simulink model "turbo_controller"  (R2025a)
settings: Solver=FixedStepAuto  StartTime=0.0  StopTime=inf  FixedStep=0.001  RelTol=1e-3
PostLoadFcn:
  | % 自动定位同目录CubeMX文件；不需要外部初始化脚本。
  | codertarget.data.setParameterValue('turbo_controller','STM32CubeMX.ProjectFile',fullfile(fileparts(get_param('turbo_controller','FileName')),'turbo_f407.ioc'));
InitFcn:
  | % 中文说明：按原控制器字段与类型创建三组接口总线；控制参数已内嵌。
  | tc_names=["EValve_Cycle" "EValve_Open" "Eblast_Cycle" "Eblast_Open" "Motor_Cycle" "Motor_Open" "EValve_Enable" "Eblast_Enable" "Motor_Enable" "SWO_Firework" "SWO_BleedAir" "EngineState" "Flag_ECUReset_Clear" "Flag_ECUReset_Save" "Flag_Reset_Enable" "Accelerator" "Nc_dem" "Nc"]; tc_types=["uint16" "uint16" "uint16" "uint16" "uint16" "uint16" "uint8" "uint8" "uint8" "uint8" "uint8" "uint8" "uint8" "uint8" "uint8" "single" "single" "single"];
  | for tc_k=1:numel(tc_names)
  |  tc_e(tc_k)=Simulink.BusElement; tc_e(tc_k).Name=char(tc_names(tc_k)); tc_e(tc_k).DataType=char(tc_types(tc_k));
  | end
  | EngineControl_Out=Simulink.Bus; EngineControl_Out.DataScope='Exported'; EngineControl_Out.Elements=tc_e;
  | clear tc_e tc_names tc_types tc_k
  | tc_names=["savedata1" "savedata2" "savedata3" "savedata4" "savedata5" "savedata6" "savedata7" "savedata8" "savedata9" "savedata10" "savedata11" "savedata12" "savedata13" "savedata14" "savedata15" "savedata16" "savedata17" "savedata18" "savedata19" "savedata20" "savedata21" "savedata22" "savedata23" "savedata24" "savedata25"]; tc_types=["single" "single" "single" "single" "single" "single" "single" "single" "single" "single" "single" "single" "single" "single" "single" "single" "single" "single" "single" "single" "single" "single" "single" "single" "single"];
  | for tc_k=1:numel(tc_names)
  |  tc_e(tc_k)=Simulink.BusElement; tc_e(tc_k).Name=char(tc_names(tc_k)); tc_e(tc_k).DataType=char(tc_types(tc_k));
  | end
  | SaveData_Out=Simulink.Bus; SaveData_Out.DataScope='Exported'; SaveData_Out.Elements=tc_e;
  | clear tc_e tc_names tc_types tc_k
  | tc_names=["senddata1" "senddata2" "senddata3" "senddata4" "senddata5" "senddata6" "senddata7" "senddata8" "senddata9" "senddata10" "senddata11" "senddata12" "senddata13" "senddata14" "senddata15" "senddata16" "senddata17" "senddata18" "senddata19" "senddata20" "senddata21" "senddata22" "senddata23" "senddata24" "senddata25" "senddata26" "senddata27" "senddata28" "senddata29"]; tc_types=["uint8" "uint8" "uint8" "uint8" "uint8" "uint8" "uint8" "uint8" "uint8" "uint8" "uint8" "uint8" "uint8" "uint8" "uint8" "uint8" "uint8" "uint8" "uint8" "uint8" "uint8" "uint8" "uint8" "uint8" "uint8" "uint8" "uint8" "uint8" "uint8"];
  | for tc_k=1:numel(tc_names)
  |  tc_e(tc_k)=Simulink.BusElement; tc_e(tc_k).Name=char(tc_names(tc_k)); tc_e(tc_k).DataType=char(tc_types(tc_k));
  | end
  | SendData_Out=Simulink.Bus; SendData_Out.DataScope='Exported'; SendData_Out.Elements=tc_e;
  | clear tc_e tc_names tc_types tc_k
  | 
  | % 以下为接口中文说明；只设置描述，不改变数值或数据类型。
  | EngineControl_Out.Description='执行控制输出（阀、电机、点火、状态及复位请求）';
  | tc_cn=["EValve_Cycle（主油阀周期计数（每计数2毫秒））" "EValve_Open（主油阀开通计数（每计数2毫秒））" "Eblast_Cycle（副油阀周期计数（每计数2毫秒））" "Eblast_Open（副油阀开通计数（每计数2毫秒））" "Motor_Cycle（起动电机周期计数）" "Motor_Open（起动电机开通计数）" "EValve_Enable（主油阀驱动使能）" "Eblast_Enable（副油阀驱动使能）" "Motor_Enable（起动电机使能）" "SWO_Firework（点火器使能（1开））" "SWO_BleedAir（引气阀使能（1开））" "EngineState（发动机状态）" "Flag_ECUReset_Clear（清除复位恢复状态请求）" "Flag_ECUReset_Save（保存复位恢复数据请求）" "Flag_Reset_Enable（处理器软件复位请求）" "Accelerator（油门／油泵给定控制量）" "Nc_dem（控制目标转速）" "Nc（发动机反馈转速（转每分））"];
  | tc_elements=EngineControl_Out.Elements;
  | for tc_k=1:numel(tc_cn)
  |  tc_elements(tc_k).Description=char(tc_cn(tc_k));
  | end
  | EngineControl_Out.Elements=tc_elements;
  | clear tc_cn tc_elements tc_k
  | SaveData_Out.Description='25项运行记录；字段含义按当前模型数据来源解释';
  | tc_cn=["savedata1（指令回显记录）" "savedata2（入口总温记录（℃））" "savedata3（电源电压记录）" "savedata4（排气温度记录（℃））" "savedata5（标定燃油压力记录）" "savedata6（副油阀占空比记录（％））" "savedata7（主油阀占空比记录（％））" "savedata8（温度修正转速记录）" "savedata9（开关输出及反馈位域）" "savedata10（物理转速记录）" "savedata11（油泵目标给定原始值）" "savedata12（起动电机占空比记录（％））" "savedata13（发动机状态码记录）" "savedata14（故障告警位域记录）" "savedata15（模型记录帧序号）" "savedata16（处理器温度记录（℃））" "savedata17（装订转速记录（沿用旧电源字段名））" "savedata18（导航高度记录）" "savedata19（飞行空速记录）" "savedata20（主阀旧记录位（恒零保留））" "savedata21（第21项保留记录（恒零））" "savedata22（保留记录项22）" "savedata23（保留记录项23）" "savedata24（保留记录项24）" "savedata25（保留记录项25）"];
  | tc_elements=SaveData_Out.Elements;
  | for tc_k=1:numel(tc_cn)
  |  tc_elements(tc_k).Description=char(tc_cn(tc_k));
  | end
  | SaveData_Out.Elements=tc_elements;
  | clear tc_cn tc_elements tc_k
  | SendData_Out.Description='29字段回传及外设命令接口；板端上位机帧只取第3至27字段';
  | tc_cn=["senddata1（回传发送允许标志（不直接上线路））" "senddata2（回传载荷长度25字节）" "senddata3（回传指令回显字节）" "senddata4（总温编码字节（℃＋80））" "senddata5（电源电压编码字节）" "senddata6（排温编码高字节）" "senddata7（排温编码低字节）" "senddata8（燃油压力编码高字节）" "senddata9（燃油压力编码低字节）" "senddata10（副油阀占空比字节（％））" "senddata11（主油阀占空比字节（％））" "senddata12（修正转速编码高字节）" "senddata13（修正转速编码低字节）" "senddata14（驱动及反馈状态位域）" "senddata15（物理转速编码高字节）" "senddata16（物理转速编码低字节）" "senddata17（油泵目标给定高字节（串口二使用））" "senddata18（油泵目标给定低字节（串口二使用））" "senddata19（起动电机占空比命令（串口一使用））" "senddata20（发动机状态码字节）" "senddata21（故障告警位域字节）" "senddata22（帧序号占位（板端另行填写））" "senddata23（处理器温度编码（℃＋50））" "senddata24（控制目标转速编码高字节）" "senddata25（控制目标转速编码低字节）" "senddata26（占位字节（板端改填实测泵速高字节））" "senddata27（占位字节（板端改填实测泵速低字节））" "senddata28（装订转速高字节（本板未发送））" "senddata29（装订转速低字节（本板未发送））"];
  | tc_elements=SendData_Out.Elements;
  | for tc_k=1:numel(tc_cn)
  |  tc_elements(tc_k).Description=char(tc_cn(tc_k));
  | end
  | SendData_Out.Elements=tc_elements;
  | clear tc_cn tc_elements tc_k
  | 
  | 
  | % FRAM模块化事务：接口类型和上电初始状态，随模型保存，无外部初始化文件。
  | clear FM_elements
  | FM_elements(1)=Simulink.BusElement;FM_elements(1).Name='phase';FM_elements(1).DataType='uint8';FM_elements(1).Dimensions=[1 1];FM_elements(1).Description='phase（当前事务阶段）';
  | FM_elements(2)=Simulink.BusElement;FM_elements(2).Name='a';FM_elements(2).DataType='uint8';FM_elements(2).Dimensions=[64 1];FM_elements(2).Description='a（启动时缓存的首区64字节）';
  | FM_elements(3)=Simulink.BusElement;FM_elements(3).Name='active';FM_elements(3).DataType='uint16';FM_elements(3).Dimensions=[1 1];FM_elements(3).Description='active（当前有效记录区地址）';
  | FM_elements(4)=Simulink.BusElement;FM_elements(4).Name='generation';FM_elements(4).DataType='uint32';FM_elements(4).Dimensions=[1 1];FM_elements(4).Description='generation（当前有效记录代号）';
  | FM_elements(5)=Simulink.BusElement;FM_elements(5).Name='record';FM_elements(5).DataType='uint8';FM_elements(5).Dimensions=[64 1];FM_elements(5).Description='record（本次冻结的待写记录）';
  | FM_elements(6)=Simulink.BusElement;FM_elements(6).Name='addr';FM_elements(6).DataType='uint16';FM_elements(6).Dimensions=[1 1];FM_elements(6).Description='addr（本次备用写入地址）';
  | FM_elements(7)=Simulink.BusElement;FM_elements(7).Name='lastSave';FM_elements(7).DataType='single';FM_elements(7).Dimensions=[1 1];FM_elements(7).Description='lastSave（上次开始保存的秒数）';
  | FM_elements(8)=Simulink.BusElement;FM_elements(8).Name='lastState';FM_elements(8).DataType='uint8';FM_elements(8).Dimensions=[1 1];FM_elements(8).Description='lastState（上次保存时的发动机状态）';
  | FM_elements(9)=Simulink.BusElement;FM_elements(9).Name='boot';FM_elements(9).DataType='boolean';FM_elements(9).Dimensions=[1 1];FM_elements(9).Description='boot（启动记录是否允许恢复）';
  | FM_elements(10)=Simulink.BusElement;FM_elements(10).Name='consumed';FM_elements(10).DataType='boolean';FM_elements(10).Dimensions=[1 1];FM_elements(10).Description='consumed（本次启动恢复通知是否已发送）';
  | FM_elements(11)=Simulink.BusElement;FM_elements(11).Name='payload';FM_elements(11).DataType='uint8';FM_elements(11).Dimensions=[20 1];FM_elements(11).Description='payload（当前20字节恢复内容）';
  | ... (+35 lines)
model workspace (MAT data in the model file):
  CRC16_Table_Reference = [0 4129 8258 12387 16516 20645 24774 28903 33032 37161 41290 45419 ... (256 elements, 256x1)]
  PE_Kaer = [0.15402 0.15402 0.12264 0.10076 0.09481 0.07601 0.07111 0.0569 0.05198 0.04926 0.05308 0.04325 ... (13 elements, 1x13)]
  PE_Nr = [21.2982 61.4260372 67.7475458 72.7394382 76.845934 80.6988798 83.8449282 86.6491912 88.9382406 89.178606 91.1938214 93.4068058 ... (13 elements, 1x13)]
  PE_Pump_Translate = 33.5999984741
  PE_RotaSpeed_Translate = 860
  PE_Taer = [0.4939154 0.4939154 0.40780982 0.34066978 0.31622756 0.30405716 0.34300244 0.26785022 0.37393554 0.23914836 0.44563948 0.31044662 ... (13 elements, 1x13)]
  PF_ACCFULLRANGE = 3360
  PF_Flag_ECUReset = 0
  PF_Flag_rx_suc = 1
  PF_Gear_Info = [40000; 45000; 50000; 55000; 57000; 59000; 60000; 61000; 61000; 61000; 61000; 61000]
  PF_K_TiaoJie = 1
  PF_Kpu = 10
  PF_MySet_Rxdata = [0 0 0 0 0 0 0 0 0 0 0 0 ... (50 elements, 50x1)]
  PF_MyUsart1_Rxdata = [0 0 0 0 0 0 0 0 0 0 0 0 ... (50 elements, 50x1)]
  PF_MyUsart2_Rxdata = [0 0 0 0 0 0 0 0 0 0 0 0 ... (50 elements, 50x1)]
  PF_Reset_Information = [0 0 0 0 0 0 0 0 0 0 0 0 ... (20 elements, 20x1)]
  PF_Sensor_X1_T4 = [0 4095]
  PF_Sensor_X2_T4 = [0 1.66666698456]
  PF_Sensor_X3_T4 = [0 504 999 1497 2010 2529 3051 3568 4076 4571 4959]
  PF_Sensor_X_P2 = [0.5 3]
  PF_Sensor_X_Poil = [0.5 3]
  PF_Sensor_X_T1t = [-50 300]
  PF_Sensor_X_Vpower = [0 3]
  PF_Sensor_X_Vpump = [0 3]
  PF_Sensor_Y1_T4 = [0 3]
  PF_Sensor_Y2_T4 = [0 5000]
  PF_Sensor_Y3_T4 = [0 100 200 300 400 500 600 700 800 900 980]
  PF_Sensor_Y_P2 = [0 1000]
  PF_Sensor_Y_Poil = [0 1000]
  PF_Sensor_Y_T1t = [-50 300]
  PF_Sensor_Y_Vpower = [0 33]
  PF_Sensor_Y_Vpump = [0 33]
  PG_CtrlMode_CloseLoop : mpt.Parameter (value not decoded)
  PG_CtrlMode_ManualAcc : mpt.Parameter (value not decoded)
  PG_CtrlMode_Origin : mpt.Parameter (value not decoded)
  PG_CtrlMode_Start : mpt.Parameter (value not decoded)
  PG_CtrlMode_Stop : mpt.Parameter (value not decoded)
  PG_ES_Clp : mpt.Parameter (value not decoded)
  PG_ES_EngStart : mpt.Parameter (value not decoded)
  PG_ES_Manual : mpt.Parameter (value not decoded)
  PG_ES_Origin : mpt.Parameter (value not decoded)
  PG_ES_Stop : mpt.Parameter (value not decoded)
  PG_Instr_BleedAirSet : mpt.Parameter (value not decoded)
  PG_Instr_CloseLoop : mpt.Parameter (value not decoded)
  PG_Instr_ECUReSet : mpt.Parameter (value not decoded)
  PG_Instr_EValveSet : mpt.Parameter (value not decoded)
  PG_Instr_EblastSet : mpt.Parameter (value not decoded)
  PG_Instr_Erase : mpt.Parameter (value not decoded)
  PG_Instr_FireWorkSet : mpt.Parameter (value not decoded)
  PG_Instr_ManualPlus : mpt.Parameter (value not decoded)
  PG_Instr_ManualrReduce : mpt.Parameter (value not decoded)
  PG_Instr_MotorSet : mpt.Parameter (value not decoded)
  PG_Instr_OilSet : mpt.Parameter (value not decoded)
  PG_Instr_SelfCheck : mpt.Parameter (value not decoded)
  PG_Instr_Start : mpt.Parameter (value not decoded)
  PG_Instr_Stop : mpt.Parameter (value not decoded)
  PG_Instr_StopZero : Simulink.Parameter (value not decoded)
  PG_Location_Air : Simulink.Parameter (value not decoded)
  PG_Location_Gnd : Simulink.Parameter (value not decoded)
  PG_ServoCtrlMode_CloseLoop : Simulink.Parameter (value not decoded)
  PG_ServoCtrlMode_CloseLoopMax : Simulink.Parameter (value not decoded)
  PG_ServoCtrlMode_CloseLoopMin : Simulink.Parameter (value not decoded)
  PG_ServoCtrlMode_ManualAcc : Simulink.Parameter (value not decoded)
  PG_ServoCtrlMode_ManualAccMax : Simulink.Parameter (value not decoded)
  PG_ServoCtrlMode_ManualAccMin : Simulink.Parameter (value not decoded)
  PG_SpeedDot_Permit : Simulink.Parameter (value not decoded)
  PL_EngineModel_Actuator = [0 10 100]
  PL_EngineModel_EngineStar_Press_P2 = [1013 1098.4 1099.144828 1099.931034 1103.613793 1162.662069 1143.793103 1131.006897 1123.186207 1117.6 1114 1111.806897 ... (127 elements, 1x127)]
  PL_EngineModel_EngineStar_RotaSpeed = [200 2000 9584 9660 10220 10240 10260 10288 10308 10368 10380 10408 ... (127 elements, 1x127)]
  PL_EngineModel_EngineStar_Temp_Exhaust = [128 129 129.1 130 131 131.1 132 133 134 134.1 135 135.1 ... (127 elements, 1x127)]
  PL_EngineModel_EngineStar_Time = [0.05 0.1 0.15 0.2 0.25 0.3 0.35 0.4 0.45 0.5 0.55 0.6 ... (127 elements, 1x127)]
  PL_EngineModel_IdleAbove_Nr = [0 21.2982 61.4260372 67.7475458 72.7394382 76.845934 80.6988798 83.8449282 86.6491912 88.9382406 89.178606 91.1938214 ... (14 elements, 1x14)]
  PL_EngineModel_IdleAbove_P2r = [0.986923266716 1.57907722675 1.81593881076 1.99358499877 2.23044658278 2.43770046879 2.65482358747 2.84233900814 3.03972366149 3.18776215149 3.25684678016 3.3950160375 ... (14 elements, 1x14)]
  PL_EngineModel_IdleAbove_Tempr = [0.0536001429337 1.07200285867 1.63301768805 1.63659103091 1.66875111667 1.72592460247 1.77595140254 1.86171163123 1.95461854565 2.03323208862 2.03323208862 2.13685903162 ... (14 elements, 1x14)]
  PL_EngineModel_IdleAbove_Ter = [0.42434128 0.42434128 0.42434128 0.30669408 0.23570008 0.22150128 0.1997974 0.23803274 0.16115638 0.24279948 0.13600422 0.31308354 ... (14 elements, 1x14)]
  PL_EngineModel_IdleAbove_Wfr = [0 10.142 23.8337 27.8905 31.9473 36.0041 40.0609 44.1177 48.1745 52.2313 52.7384 56.7952 ... (14 elements, 1x14)]
  PL_EngineModel_Press_P2 = [400 400 400 400 400 400 400 400 400 400]
  PL_EngineModel_Rotaspeed = [0 20000 96400]
  PL_EngineModel_Temp_Exhaust = [500 500 500 500 500 500 500 500 500 500]
  PL_Kaer = [0.1 0.1 0.1 0.1 0.1 0.1]
  PL_Nr = [50 60 70 80 90 100]
  PL_Taer = [0.1 0.1 0.1 0.1 0.1 0.1]
  Sig : Simulink.Signal (value not decoded)
  Ts_ms : Simulink.Parameter (value not decoded)
  false : Simulink.Parameter (value not decoded)
  true : Simulink.Parameter (value not decoded)
symbols that are objects in the model workspace (value not decoded): PG_CtrlMode_CloseLoop, PG_CtrlMode_ManualAcc, PG_CtrlMode_Origin, PG_CtrlMode_Start, PG_CtrlMode_Stop, PG_ES_Clp, PG_ES_EngStart, PG_ES_Manual, PG_ES_Origin, PG_ES_Stop, PG_Instr_BleedAirSet, PG_Instr_CloseLoop, PG_Instr_EblastSet, PG_Instr_ECUReSet, PG_Instr_Erase, PG_Instr_EValveSet, PG_Instr_FireWorkSet, PG_Instr_ManualPlus, PG_Instr_ManualrReduce, PG_Instr_MotorSet, PG_Instr_OilSet, PG_Instr_SelfCheck, PG_Instr_Start, PG_Instr_Stop, PG_Instr_StopZero, PG_ServoCtrlMode_CloseLoop, PG_ServoCtrlMode_CloseLoopMax, PG_ServoCtrlMode_CloseLoopMin, PG_ServoCtrlMode_ManualAcc, PG_ServoCtrlMode_ManualAccMax, PG_ServoCtrlMode_ManualAccMin, Ts_ms
libraries: simulink x97, stm32blockslib x10, stm32f4xxblockslib x8
(part 18 of 26)

== system turbo_controller/BoardInput_输入换算与协议解析/In03_Pump（油泵回包预留校验）/Receive（逐字节组帧与保持有效结果）_353/Step01_取字节与循环控制 ==
  note: 第一步：只处理本批收到的字节
      |
      | 接收数组最多64项，Count是这次新收到的数量，Loop给出从1开始的Index。Byte=Rx(Index)，Active=
      | (Index≤Count)。
      |
      | 处理到Index≥Count或Index=64，就把下一循环序号设65，使Loop退出；否则下一序号=Index+1。Coun
      | t=3只处理第1～3项；Count=0时仍走一次无效项保持路径，但不会把数组旧值加入帧。
      |
      | 输出Byte和Active给组帧步骤，下一序号反馈Loop。这里不识别帧头，不作CRC，不把Index当作跨批收
      | 帧位置。
  输入1_本批循环序号 : Inport
  输入2_本批有效字节数 : Inport  Port=2
  输入3_本批接收数组 : Inport  Port=3
  Active（本项在有效范围内）_242 : RelationalOperator  Operator=<=  OutDataTypeStr=boolean  RndMeth=Simplest  InputSameDT=off
  Add（加减运算）_249 : Sum  SaturateOnIntegerOverflow=on  OutDataTypeStr=Inherit: Same as first input
  AtLimit（达到处理上限）_245 : RelationalOperator  Operator===  OutDataTypeStr=boolean  RndMeth=Simplest  InputSameDT=off
  Constant（常量）_244 : Constant  Value=64  OutDataTypeStr=uint32
  Constant（常量）_247 : Constant  Value=65  OutDataTypeStr=uint32
  Constant（常量）_248 : Constant  OutDataTypeStr=uint32
  CurrentByte（按接收顺序取字节）_251 : Selector  InputPortWidth=64  IndexOptions=Index vector (port)  Indices=1  OutputSizes=1
  Last（本周期最后一项）_246 : Logic  Operator=OR  IconShape=distinctive  AllPortsSameDT=off  OutDataTypeStr=boolean
  NextIndex（处理下一项或结束）_250 : Switch  Criteria=u2 ~= 0  SaturateOnIntegerOverflow=off  InputSameDT=off
  ReceivedAll（已处理所有有效项）_243 : RelationalOperator  OutDataTypeStr=boolean  RndMeth=Simplest  InputSameDT=off
  输出1_本项字节 : Outport
  输出2_本项字节有效 : Outport  Port=2
  输出3_下一循环序号 : Outport  Port=3
  wires:
  NextIndex（处理下一项或结束）_250/1 -> 输出3_下一循环序号/1
  Active（本项在有效范围内）_242/1 -> 输出2_本项字节有效/1
  CurrentByte（按接收顺序取字节）_251/1 -> 输出1_本项字节/1
  Add（加减运算）_249/1 -> NextIndex（处理下一项或结束）_250/3
  Last（本周期最后一项）_246/1 -> NextIndex（处理下一项或结束）_250/2
  Constant（常量）_247/1 -> NextIndex（处理下一项或结束）_250/1
  AtLimit（达到处理上限）_245/1 -> Last（本周期最后一项）_246/2
  ReceivedAll（已处理所有有效项）_243/1 -> Last（本周期最后一项）_246/1
  输入3_本批接收数组/1 -> CurrentByte（按接收顺序取字节）_251/1
  Constant（常量）_244/1 -> AtLimit（达到处理上限）_245/2
  Constant（常量）_248/1 -> Add（加减运算）_249/2
  输入2_本批有效字节数/1 -> Active（本项在有效范围内）_242/2, ReceivedAll（已处理所有有效项）_243/2
  输入1_本批循环序号/1 -> Add（加减运算）_249/1, Active（本项在有效范围内）_242/1, AtLimit（达到处理上限）_245/1, ReceivedAll（已处理所有有效项）_243/1, CurrentByte（按接收顺序取字节）_251/2

== system turbo_controller/BoardInput_输入换算与协议解析/In03_Pump（油泵回包预留校验）/Receive（逐字节组帧与保持有效结果）_353/Step02_拼帧并保存半帧 ==
  note: 第二步：跨多次接收保存半帧
      |
      | 将本项字节、有效标志、上次候选缓存和上次收帧Position交给Collect。Collect识别AA55并逐项填满
      | 22字节，具体规则已在其内部再拆成五步。
      |
      | 更新后的缓存和Position经原数据类型转换，送回两条记忆块；所以第一次只收到一半，下一批还能接
      | 着填，不必从头找AA。输出候选帧与“本字节刚收齐”，交第三步校验。
      |
      | 候选缓存不等于已接受结果。即使旧缓存里已经有完整内容，没有本次收齐事件也不能再次接受它。这
      | 里的记忆按原循环节奏推进，没有增加一个额外的采样周期等待。
  输入1_本项字节 : Inport
  输入2_本项字节有效 : Inport  Port=2
  Buffer（跨周期收帧缓存）_252 : UnitDelay  InitialCondition=uint8(zeros(22,1))  SampleTime=-1  HasFrameUpgradeWarning=on
  Collect（帧头识别与缓存推进）_293 : Subsystem  Description=|
      | 逐字节组帧：本页只做“找帧头、存字节、推进位置”
      | 
      | 固定帧长为22字节，帧头是十六进制AA、55。输入为上一份候选缓存、已收字节数Position、本次Byte和本字节有效Active。输出为更新缓存、下一次使用的Position和本次收齐事件Complete。
      | 
      | Position不是本批接收数组的序号：0表示还在找AA，1表示已见AA、正在等55，2～21表示头部已确认、继续收后面的内容。跨调用的记忆由外层Step02保存，本页根据输入计算一次更新。
      | 
      | 按五步看：
      | 1 判断当前是否在等AA或55，以及字节是否匹配。
      | 2 决定这个字节应不应该进入候选缓存。
      | 3 算出本次写入位置Position+1，判断是否达到22。
      | 4 允许写入才更新对应一项，否则保留原缓存。
      | 5 按找头、重同步、收齐和无效字节规则，决定下一位置及Complete。
      | 
      | 例：AA→AA→55时，第二个AA保留继续等55的机会，不当作第二帧头写入；头确认后，后续数据即使也是AA或55，仍按普通数据收下。无效字节不推进位置，也不发收齐事件。
      | 
      | Complete仅表示候选帧刚拼满，不表示校验通过；外面的校验步骤还会检查内容。这里没有重写协议或增加等待时间，五步在同一次字节处理内完成。
  Position（已收到的字节数）_253 : UnitDelay  InitialCondition=uint16(0)  SampleTime=-1  HasFrameUpgradeWarning=on
  Store_uint16（按十六位无符号数保存状态）_536715 : DataTypeConversion  Description=为反馈回路显式指定原程序的状态类型，保持原状态更新节拍。  OutDataTypeStr=uint16  RndMeth=Round
  Store_uint8（按八位无符号数保存状态）_536714 : DataTypeConversion  Description=为反馈回路显式指定原程序的状态类型，保持原状态更新节拍。  OutDataTypeStr=uint8  RndMeth=Round
  输出1_本字节刚收齐 : Outport
  输出2_候选帧缓存 : Outport  Port=2
  wires:
  Collect（帧头识别与缓存推进）_293/3(Complete（本字节组成完整帧）_292) -> 输出1_本字节刚收齐/1  "Collect（帧头识别与缓存推进）"
  Collect（帧头识别与缓存推进）_293/1(Buffer（更新后的帧缓存）_290) -> 输出2_候选帧缓存/1, Store_uint8（按八位无符号数保存状态）_536714/1  "Collect（帧头识别与缓存推进）"
  Collect（帧头识别与缓存推进）_293/2(Position（下次接收位置）_291) -> Store_uint16（按十六位无符号数保存状态）_536715/1  "Collect（帧头识别与缓存推进）"
  Store_uint16（按十六位无符号数保存状态）_536715/1 -> Position（已收到的字节数）_253/1
  输入2_本项字节有效/1 -> Collect（帧头识别与缓存推进）_293/4(Active（当前字节有效）_257)
  输入1_本项字节/1 -> Collect（帧头识别与缓存推进）_293/3(Byte（当前字节）_256)
  Position（已收到的字节数）_253/1 -> Collect（帧头识别与缓存推进）_293/2(Position（已收字节数）_255)
  Buffer（跨周期收帧缓存）_252/1 -> Collect（帧头识别与缓存推进）_293/1(Buffer（上次收帧缓存）_254)
  Store_uint8（按八位无符号数保存状态）_536714/1 -> Buffer（跨周期收帧缓存）_252/1

== system turbo_controller/BoardInput_输入换算与协议解析/In03_Pump（油泵回包预留校验）/Receive（逐字节组帧与保持有效结果）_353/Step03_收齐且校验通过才接受 ==
  note: 第三步：刚收齐且CRC通过，才接受新帧
      |
      | Complete表示这一项字节刚把22字节补齐，先按原类型传给Verify触发校验。Verify对第6～20字节计
      | 算CRC16，分别与第21、22字节的高、低校验字节比较。
      |
      | 最后Accepted=Complete AND Verify通过。这样未收齐的数据不会被采用，Verify上一帧保留的通过状
      | 态也不会在没有新Complete时重新接收旧帧。
      |
      | CRC初值、表和覆盖范围保留原设置。校验失败只让本次Accepted为假；后面的批次统计继续看这一批
      | 有没有其他有效帧。本处不作反馈比例换算，不直接生成驱动命令。
  输入1_本字节刚收齐 : Inport
  输入2_候选帧缓存 : Inport  Port=2
  Accepted（本字节完成一帧有效数据）_345 : Logic  IconShape=distinctive  AllPortsSameDT=off  OutDataTypeStr=boolean
  Cast（数据类型转换）_343 : DataTypeConversion  OutDataTypeStr=uint32  RndMeth=Round
  Verify（完整帧校验）_344 : Subsystem  Description=|
      | 输入侧预留22字节油泵帧怎样核对CRC
      | 
      | Collect送来的是候选完整帧，本模块只在Complete有效时执行校验。内部取协议指定的待校验字节段，送CRC16逐字节计算，并取出帧尾携带的两个CRC字节。
      | 
      | 16位计算结果分为高低两部分：高字节=floor(CRC/256)，低字节=bitand(CRC,255)。分别与帧中对应位置比较，两项都一致才给出有效结果。
      | 
      | 比如计算CRC为十六进制1234，协议中的CRC高字节必须是12、低字节必须是34；顺序反过来也不能通过。CRC覆盖范围由本页Selector的固定索引决定，不应把帧头或尾部CRC自身随意加入。
      | 
      | 输出交给Receive，与“这一轮确实刚收齐一帧”共同决定是否更新反馈。不完整或校验错误时，外层保留最近有效结果。
      | 
      | 本实例CRC覆盖第6～20字节，与第21、22字节的CRC比较。
  输出1_本字节接受有效帧 : Outport
  wires:
  Accepted（本字节完成一帧有效数据）_345/1 -> 输出1_本字节接受有效帧/1
  输入2_候选帧缓存/1 -> Verify（完整帧校验）_344/2(Frame（完整候选帧）_296)
  Cast（数据类型转换）_343/1 -> Verify（完整帧校验）_344/1(Complete（完整帧执行一次）_294)
  Verify（完整帧校验）_344/1(Valid（校验是否通过）_342) -> Accepted（本字节完成一帧有效数据）_345/2  "Verify（完整帧校验）"
  输入1_本字节刚收齐/1 -> Accepted（本字节完成一帧有效数据）_345/1, Cast（数据类型转换）_343/1

== system turbo_controller/BoardInput_输入换算与协议解析/In03_Pump（油泵回包预留校验）/Receive（逐字节组帧与保持有效结果）_353/Step04_统计本批是否有有效帧 ==
  note: 第四步：统计本批有没有接受过有效帧
      |
      | 根据Loop的Index判断是不是本批第一项。第一项先把累计结果视为false，后续项继续采用Seen记忆；
      | 再把这个累计结果与本项Accepted作OR。
      |
      | 只要这一批某项收齐并校验通过，后面即使是普通字节或无效帧，批次结果仍保持true；下一批会在第
      | 一项重新统计。它不是跨所有批次永久锁存的有效标志。
      |
      | 例如本批先坏帧、后好帧，最后输出true；整批没有好帧则false。此分支只输出校验统计，不计算泵
      | 速，也没有0.875/0.125滤波，不能与BoardOutput内的实际泵反馈路径混淆。
  输入1_本字节接受有效帧 : Inport
  输入2_本批循环序号 : Inport  Port=2
  AnyValid（本次存在有效帧）_351 : Logic  Operator=OR  IconShape=distinctive  AllPortsSameDT=off  OutDataTypeStr=boolean
  BeginTick（每毫秒重新统计）_350 : Switch  Criteria=u2 ~= 0  SaturateOnIntegerOverflow=off  InputSameDT=off
  Compare（比较）_348 : RelationalOperator  Operator===  OutDataTypeStr=boolean  RndMeth=Simplest  InputSameDT=off
  Constant（常量）_347 : Constant  OutDataTypeStr=uint32
  Constant（常量）_349 : Constant  Value=false  OutDataTypeStr=boolean
  Seen（本次是否见过有效帧）_346 : UnitDelay  InitialCondition=logical(0)  SampleTime=-1  HasFrameUpgradeWarning=on
  Store_boolean（按逻辑值保存状态）_536720 : DataTypeConversion  Description=为反馈回路显式指定原程序的状态类型，保持原状态更新节拍。  OutDataTypeStr=boolean  RndMeth=Round
  输出1_本批出现过有效帧 : Outport
  wires:
  AnyValid（本次存在有效帧）_351/1 -> 输出1_本批出现过有效帧/1, Store_boolean（按逻辑值保存状态）_536720/1
  Store_boolean（按逻辑值保存状态）_536720/1 -> Seen（本次是否见过有效帧）_346/1
  Constant（常量）_347/1 -> Compare（比较）_348/2
  输入2_本批循环序号/1 -> Compare（比较）_348/1
  Seen（本次是否见过有效帧）_346/1 -> BeginTick（每毫秒重新统计）_350/3
  Compare（比较）_348/1 -> BeginTick（每毫秒重新统计）_350/2
  Constant（常量）_349/1 -> BeginTick（每毫秒重新统计）_350/1
  输入1_本字节接受有效帧/1 -> AnyValid（本次存在有效帧）_351/2
  BeginTick（每毫秒重新统计）_350/1 -> AnyValid（本次存在有效帧）_351/1

== system turbo_controller/BoardInput_输入换算与协议解析/In04_Capture（捕获间隔缓存）/Step03_计算间隔并更新环形缓存/Step01_计算回卷后的脉冲间隔 ==
  note: 第一步：把16位捕获读数换成正向间隔
      |
      | 先转换当前与上次读数的类型，避免直接用无符号数相减造成负差丢失。再计算：
      | 间隔=mod(本次Capture-上次Previous,65536)。
      |
      | 当前配置每个计数为1微秒。例：上次1000、当前2000，得到1000微秒；上次65530、当前4，得到10微
      | 秒。65536来自16位计数器的一个完整回卷周期。
      |
      | 本步骤只产生候选间隔，不检查Active，也不写缓存。回卷差分只保留模65536的结果，并没有额外累
      | 计跨越多个完整回卷的时间。
      |
      | 初始Previous沿用原模型的0，所以第一条正读数会相对0求差；本次拆分没有新增“第一脉冲只初始化
      | ”的规则。
  输入1_本项捕获读数 : Inport
  输入2_上一捕获读数 : Inport  Port=2
  Cast（数据类型转换）_382 : DataTypeConversion  OutDataTypeStr=double  RndMeth=Round
  Cast（数据类型转换）_383 : DataTypeConversion  OutDataTypeStr=double  RndMeth=Round
  Cast（数据类型转换）_387 : DataTypeConversion  OutDataTypeStr=uint32  RndMeth=Floor
  Constant（常量）_385 : Constant  Value=65536  OutDataTypeStr=double
  Difference（捕获计数差）_384 : Sum  Inputs=+-  SaturateOnIntegerOverflow=on  OutDataTypeStr=Inherit: Same as first input
  Wrap16（十六位计数回卷差分）_386 : Math  Operator=mod
  输出1_回卷后的脉冲间隔 : Outport
  wires:
  Cast（数据类型转换）_387/1 -> 输出1_回卷后的脉冲间隔/1
  Constant（常量）_385/1 -> Wrap16（十六位计数回卷差分）_386/2
  Difference（捕获计数差）_384/1 -> Wrap16（十六位计数回卷差分）_386/1
  Cast（数据类型转换）_383/1 -> Difference（捕获计数差）_384/2
  Cast（数据类型转换）_382/1 -> Difference（捕获计数差）_384/1
  Wrap16（十六位计数回卷差分）_386/1 -> Cast（数据类型转换）_387/1
  输入2_上一捕获读数/1 -> Cast（数据类型转换）_383/1
  输入1_本项捕获读数/1 -> Cast（数据类型转换）_382/1

== system turbo_controller/BoardInput_输入换算与协议解析/In04_Capture（捕获间隔缓存）/Step03_计算间隔并更新环形缓存/Step02_判断间隔是否有效 ==
  note: 第二步：决定这个间隔能否新增一条记录
      |
      | 允许保存=Active AND 间隔>0。
      |
      | Active说明本项确实属于本批新捕获，间隔>0排除重复读数。例：本次捕获和上次相同，间隔0，虽然A
      | ctive为真，也不新增间隔、不推进环形位置、不增加数量、不刷新最近有效时间。
      |
      | 没有有效新项时，即使候选差分非0，也不采用。这个许可送最后的提交步骤；本步骤自身没有记忆，
      | 也不判断转速是否超限。
  输入1_回卷后的脉冲间隔 : Inport
  输入2_本项捕获有效 : Inport  Port=2
  Constant（常量）_388 : Constant  Value=0  OutDataTypeStr=uint32
  Nonzero（零间隔丢弃）_389 : RelationalOperator  Operator=>  OutDataTypeStr=boolean  RndMeth=Simplest  InputSameDT=off
  Valid（可保存的有效间隔）_390 : Logic  IconShape=distinctive  AllPortsSameDT=off  OutDataTypeStr=boolean
  输出1_允许保存正间隔 : Outport
  wires:
  Valid（可保存的有效间隔）_390/1 -> 输出1_允许保存正间隔/1
  Nonzero（零间隔丢弃）_389/1 -> Valid（可保存的有效间隔）_390/2
  输入2_本项捕获有效/1 -> Valid（可保存的有效间隔）_390/1
  Constant（常量）_388/1 -> Nonzero（零间隔丢弃）_389/2
  输入1_回卷后的脉冲间隔/1 -> Nonzero（零间隔丢弃）_389/1

== system turbo_controller/BoardInput_输入换算与协议解析/In04_Capture（捕获间隔缓存）/Step03_计算间隔并更新环形缓存/Step03_生成缓存写入候选值 ==
  note: 第三步：准备一份只改一项的缓存候选值
      |
      | 按当前Index，把本次间隔写进旧Ring对应的位置，其余九项保留。Index是1～10的环形写入位置，不
      | 是本批捕获数组的序号。
      |
      | 例：Index=4、间隔1000，则候选数组只把第4项换成1000。即使第二步不允许保存，这里也可算出候选
      | 数组；最终会由第六步选择旧缓存，候选值不会生效。
      |
      | 这里的Assignment不增加数组长度，不求平均，也不清空其他项。
  输入1_回卷后的脉冲间隔 : Inport
  输入2_旧十项间隔缓存 : Inport  Port=2
  输入3_当前环形写入位置 : Inport  Port=3
  Cast（数据类型转换）_391 : DataTypeConversion  OutDataTypeStr=single  RndMeth=Round
  WriteRing（写入最近十个间隔）_392 : Assignment  DiagnosticForDimensions=Warning  IndexOptions=Index vector (port)  Indices=1  OutputSizes=1
  输出1_候选十项间隔缓存 : Outport
  wires:
  WriteRing（写入最近十个间隔）_392/1 -> 输出1_候选十项间隔缓存/1
  输入3_当前环形写入位置/1 -> WriteRing（写入最近十个间隔）_392/3
  Cast（数据类型转换）_391/1 -> WriteRing（写入最近十个间隔）_392/2
  输入2_旧十项间隔缓存/1 -> WriteRing（写入最近十个间隔）_392/1
  输入1_回卷后的脉冲间隔/1 -> Cast（数据类型转换）_391/1

== system turbo_controller/BoardInput_输入换算与协议解析/In04_Capture（捕获间隔缓存）/Step03_计算间隔并更新环形缓存/Step04_计算下次环形写入位置 ==
  note: 第四步：准备下一次应覆盖的环形位置
      |
      | 候选下一位置=mod(本次Index,10)+1。
      |
      | Index=1得到2，Index=9得到10，Index=10得到1。这样十项写满后继续从第1项覆盖最旧记录。
      |
      | 本步骤只算候选位置；只有第六步收到保存许可才采用它。零间隔或无效捕获不会因为这里已经算出下
      | 一位置就推进缓存。
  输入1_当前环形写入位置 : Inport
  Add（加减运算）_397 : Sum  SaturateOnIntegerOverflow=on  OutDataTypeStr=Inherit: Same as first input
  Cast（数据类型转换）_393 : DataTypeConversion  OutDataTypeStr=double  RndMeth=Round
  Constant（常量）_394 : Constant  Value=10  OutDataTypeStr=double
  Constant（常量）_396 : Constant  OutDataTypeStr=double
  Modulo（取余）_395 : Math  Operator=mod
  NextSlot（写满十项后回到第一项）_398 : DataTypeConversion  OutDataTypeStr=uint8  RndMeth=Floor
  输出1_候选下次写入位置 : Outport
  wires:
  NextSlot（写满十项后回到第一项）_398/1 -> 输出1_候选下次写入位置/1
  Add（加减运算）_397/1 -> NextSlot（写满十项后回到第一项）_398/1
  Constant（常量）_394/1 -> Modulo（取余）_395/2
  Cast（数据类型转换）_393/1 -> Modulo（取余）_395/1
  输入1_当前环形写入位置/1 -> Cast（数据类型转换）_393/1
  Constant（常量）_396/1 -> Add（加减运算）_397/2
  Modulo（取余）_395/1 -> Add（加减运算）_397/1

== system turbo_controller/BoardInput_输入换算与协议解析/In04_Capture（捕获间隔缓存）/Step03_计算间隔并更新环形缓存/Step05_计算已保存间隔数量 ==
  note: 第五步：准备累计有效间隔数量
      |
      | 候选数量=min(旧Count+1,10)。
      |
      | 未填满时，每接受一个正间隔增加1；达到10后保持10。例：旧数量8得到候选9，旧数量10仍得到10。
      | 数量到10不会让后续数据停止写入，环形位置仍继续轮转覆盖。
      |
      | 本步骤不是统计本批有几个捕获。它计算缓存有效条数的候选值，只有第六步有保存许可才提交；否则
      | 继续旧Count。
  输入1_累计有效间隔数 : Inport
  Add（加减运算）_401 : Sum  SaturateOnIntegerOverflow=on  OutDataTypeStr=Inherit: Same as first input
  Constant（常量）_399 : Constant  Value=10  OutDataTypeStr=uint8
  Constant（常量）_400 : Constant  OutDataTypeStr=uint8
  Filled（有效个数最多十项）_402 : MinMax  Inputs=2
  输出1_候选有效间隔数量 : Outport
  wires:
  Filled（有效个数最多十项）_402/1 -> 输出1_候选有效间隔数量/1
  Add（加减运算）_401/1 -> Filled（有效个数最多十项）_402/2
  Constant（常量）_399/1 -> Filled（有效个数最多十项）_402/1
  Constant（常量）_400/1 -> Add（加减运算）_401/2
  输入1_累计有效间隔数/1 -> Add（加减运算）_401/1

== system turbo_controller/BoardInput_输入换算与协议解析/In04_Capture（捕获间隔缓存）/Step03_计算间隔并更新环形缓存/Step06_有效才提交并更新时间 ==
  note: 第六步：按许可提交候选状态，并记录新鲜程度
      |
      | 分别选择两类状态：
      | Previous：Active为真就采用当前Capture，否则保持旧Previous。
      | Ring、Index、Count、LastTime：只有第二步允许保存时，才采用第三～五步候选值，并把LastTime更
      | 新为当前Seconds；否则全部保持旧值。
      |
      | 例：有效捕获但与上次相同，Previous仍更新到当前读数，其他四项不变。这种情况下不会伪造一条0
      | 间隔，也不会让后面的超时判断误以为又收到了一条有效间隔。
      |
      | LastTime记录的是本批处理时刻，单位秒；同一批多个捕获共用这一时刻。它不等同于每个脉冲精确的
      | 硬件到达时刻，精确间隔来自计数差分。
      |
      | 五项输出交外层记忆。本处没有新增延迟，没有直接输出转速，也不负责选择电机反馈或捕获测速。
  输入1_本项捕获读数 : Inport
  输入2_当前处理时刻_秒 : Inport  Port=2
  输入3_本项捕获有效 : Inport  Port=3
  输入4_上一捕获读数 : Inport  Port=4
  输入5_候选十项间隔缓存 : Inport  Port=5
  输入6_允许保存正间隔 : Inport  Port=6
  输入7_旧十项间隔缓存 : Inport  Port=7
  输入8_候选下次写入位置 : Inport  Port=8
  输入9_当前环形写入位置 : Inport  Port=9
  输入10_候选有效间隔数量 : Inport  Port=10
  输入11_累计有效间隔数 : Inport  Port=11
  输入12_上次有效间隔时刻 : Inport  Port=12
  Cast（数据类型转换）_403 : DataTypeConversion  OutDataTypeStr=uint32  RndMeth=Round
  Cast（数据类型转换）_412 : DataTypeConversion  OutDataTypeStr=single  RndMeth=Round
  Select（按条件选择）_{404,406,408,410,413} (5 alike) : Switch  Criteria=u2 ~= 0  SaturateOnIntegerOverflow=off  InputSameDT=off
  输出1_下一差分基准 : Outport
  输出2_更新后的十项间隔 : Outport  Port=2
  输出3_下一环形写入位置 : Outport  Port=3
  输出4_更新后的有效间隔数 : Outport  Port=4
  输出5_最近有效间隔处理时刻 : Outport  Port=5
  wires:
  输入1_本项捕获读数/1 -> Cast（数据类型转换）_403/1
  输入2_当前处理时刻_秒/1 -> Cast（数据类型转换）_412/1
  Cast（数据类型转换）_403/1 -> Select（按条件选择）_404/1
  输入3_本项捕获有效/1 -> Select（按条件选择）_404/2
  输入4_上一捕获读数/1 -> Select（按条件选择）_404/3
  输入9_当前环形写入位置/1 -> Select（按条件选择）_408/3
  输入5_候选十项间隔缓存/1 -> Select（按条件选择）_406/1
  Select（按条件选择）_406/1 -> 输出2_更新后的十项间隔/1
  输入11_累计有效间隔数/1 -> Select（按条件选择）_410/3
  输入7_旧十项间隔缓存/1 -> Select（按条件选择）_406/3
  Cast（数据类型转换）_412/1 -> Select（按条件选择）_413/1
  Select（按条件选择）_404/1 -> 输出1_下一差分基准/1
  输入12_上次有效间隔时刻/1 -> Select（按条件选择）_413/3
  输入10_候选有效间隔数量/1 -> Select（按条件选择）_410/1
  输入6_允许保存正间隔/1 -> Select（按条件选择）_410/2, Select（按条件选择）_408/2, Select（按条件选择）_413/2, Select（按条件选择）_406/2
  输入8_候选下次写入位置/1 -> Select（按条件选择）_408/1
  Select（按条件选择）_413/1 -> 输出5_最近有效间隔处理时刻/1
  Select（按条件选择）_408/1 -> 输出3_下一环形写入位置/1
  Select（按条件选择）_410/1 -> 输出4_更新后的有效间隔数/1

== system turbo_controller/BoardInput_输入换算与协议解析/In05_Speed（转速来源选择与滤波）/CaptureSpeed（去极值估算转速）_19/Step01_选出有效间隔 ==
  note: 第一步：标出前n个有效位置，求和时把其他位置变0
      |
      | 缓存固定十项，但刚开始未必填满。将序号1～10分别与Count比较，序号≤Count才标记为有效。
      |
      | 求和用的数组：有效位置保留原间隔，无效位置填0。与此同时把有效位置掩码送下一步，用于寻找真
      | 正有效项中的最大值和最小值。
      |
      | 例：Count=3，缓存[1000,1100,900,0,…]，求和数组只采用前三项，后七项不作为测量。Count是间隔
      | 条数，不是时间，也不是每转脉冲数。
      |
      | 本步骤不改写原缓存，只生成本次计算用的数据与掩码。
  输入1_有效间隔条数 : Inport
  输入2_原十项间隔缓存 : Inport  Port=2
  Cast（数据类型转换）_447 : DataTypeConversion  OutDataTypeStr=uint32  RndMeth=Round
  Constant（常量）_449 : Constant  Value=zeros(10,1)  OutDataTypeStr=single
  Indices（十项缓存的序号）_446 : Constant  Value=(1:10)'  OutDataTypeStr=uint32
  ValidSlots（只用前面有效的项）_448 : RelationalOperator  Operator=<=  OutDataTypeStr=boolean  RndMeth=Simplest  InputSameDT=off
  ValidValues（无效项按零参加求和）_450 : Switch  Criteria=u2 ~= 0  SaturateOnIntegerOverflow=off  InputSameDT=off
  输出1_有效位置掩码 : Outport
  输出2_无效项已清零的求和数据 : Outport  Port=2
  wires:
  ValidValues（无效项按零参加求和）_450/1 -> 输出2_无效项已清零的求和数据/1
  Constant（常量）_449/1 -> ValidValues（无效项按零参加求和）_450/3
  ValidSlots（只用前面有效的项）_448/1 -> 输出1_有效位置掩码/1, ValidValues（无效项按零参加求和）_450/2
  输入2_原十项间隔缓存/1 -> ValidValues（无效项按零参加求和）_450/1
  Cast（数据类型转换）_447/1 -> ValidSlots（只用前面有效的项）_448/2
  Indices（十项缓存的序号）_446/1 -> ValidSlots（只用前面有效的项）_448/1
  输入1_有效间隔条数/1 -> Cast（数据类型转换）_447/1

== system turbo_controller/BoardInput_输入换算与协议解析/In05_Speed（转速来源选择与滤波）/CaptureSpeed（去极值估算转速）_19/Step02_去掉最大最小再求和 ==
  note: 第二步：去掉一个最大间隔和一个最小间隔
      |
      | 先对第一步的求和数组求总和。找最大值时，无效位置用0占位；找最小值时，无效位置用single最大
      | 有限值占位，避免未填满缓存的0被误当作最小有效间隔。
      |
      | S=有效间隔总和-最大有效间隔-最小有效间隔。
      | 例：[900,1000,1100]的总和3000，去掉1100和900，S=1000；剩下一项用于估速。若十项都是1000，去
      | 掉其中两项，S=8000。
      |
      | 每种极值只减一项；即使有多个相同最大值，也不是全部删除。这里求的是剩余间隔总和，还没有除以
      | n-2；第四步会把剩余项数并入转速公式。
  输入1_原十项间隔缓存 : Inport
  输入2_有效位置掩码 : Inport  Port=2
  输入3_无效项已清零的求和数据 : Inport  Port=3
  Constant（常量）_452 : Constant  Value=0  OutDataTypeStr=single
  Constant（常量）_455 : Constant  Value=realmax('single')  OutDataTypeStr=single
  Maximum（去掉一个最大间隔）_454 : MinMax  Function=max
  Minimum（去掉一个最小间隔）_457 : MinMax
  Select（按条件选择）_453 : Switch  Criteria=u2 ~= 0  SaturateOnIntegerOverflow=off  InputSameDT=off
  Select（按条件选择）_456 : Switch  Criteria=u2 ~= 0  SaturateOnIntegerOverflow=off  InputSameDT=off
  Sum（有效间隔总和）_451 : Sum  Inputs=+  OutDataTypeStr=single  AccumDataTypeStr=single
  TrimmedSum（去掉一个最大值和一个最小值）_458 : Sum  Inputs=+--  SaturateOnIntegerOverflow=on  OutDataTypeStr=Inherit: Same as first input
  输出1_去极值后间隔总和 : Outport
  wires:
  输入1_原十项间隔缓存/1 -> Select（按条件选择）_453/1, Select（按条件选择）_456/1
  输入2_有效位置掩码/1 -> Select（按条件选择）_456/2, Select（按条件选择）_453/2
  Constant（常量）_452/1 -> Select（按条件选择）_453/3
  Constant（常量）_455/1 -> Select（按条件选择）_456/3
  输入3_无效项已清零的求和数据/1 -> Sum（有效间隔总和）_451/1
  Select（按条件选择）_453/1 -> Maximum（去掉一个最大间隔）_454/1
  Select（按条件选择）_456/1 -> Minimum（去掉一个最小间隔）_457/1
  Sum（有效间隔总和）_451/1 -> TrimmedSum（去掉一个最大值和一个最小值）_458/1
  Maximum（去掉一个最大间隔）_454/1 -> TrimmedSum（去掉一个最大值和一个最小值）_458/2
  TrimmedSum（去掉一个最大值和一个最小值）_458/1 -> 输出1_去极值后间隔总和/1
  Minimum（去掉一个最小间隔）_457/1 -> TrimmedSum（去掉一个最大值和一个最小值）_458/3

== system turbo_controller/BoardInput_输入换算与协议解析/In05_Speed（转速来源选择与滤波）/CaptureSpeed（去极值估算转速）_19/Step03_检查分母并防止除零 ==
  note: 第三步：判断去极值后的总和能否作分母
      |
      | Valid=(S>0)。有效时把S交给下一步；无效时，内部改用1作为安全分母，避免除零。
      |
      | 安全分母1只是防止算术错误，不能表示测量间隔为1微秒。Valid为假时，后面的数值输出不可单独当
      | 作有效转速。
      |
      | 本步骤也不判断Count≥3。这个数量条件在外层Status；只有数量、分母和时间条件都满足，外层才会
      | 采用捕获估速。
  输入1_去极值后间隔总和 : Inport
  Constant（常量）_459 : Constant  Value=0  OutDataTypeStr=single
  Constant（常量）_461 : Constant  OutDataTypeStr=single
  Positive（分母必须大于零）_460 : RelationalOperator  Operator=>  OutDataTypeStr=boolean  RndMeth=Simplest  InputSameDT=off
  SafeDenominator（无效时避免除零）_462 : Switch  Criteria=u2 ~= 0  SaturateOnIntegerOverflow=off  InputSameDT=off
  输出1_用于计算的安全分母 : Outport
  输出2_分母为正 : Outport  Port=2
  wires:
  SafeDenominator（无效时避免除零）_462/1 -> 输出1_用于计算的安全分母/1
  Constant（常量）_461/1 -> SafeDenominator（无效时避免除零）_462/3
  Positive（分母必须大于零）_460/1 -> SafeDenominator（无效时避免除零）_462/2, 输出2_分母为正/1
  Constant（常量）_459/1 -> Positive（分母必须大于零）_460/2
  输入1_去极值后间隔总和/1 -> SafeDenominator（无效时避免除零）_462/1, Positive（分母必须大于零）_460/1

== system turbo_controller/BoardInput_输入换算与协议解析/In05_Speed（转速来源选择与滤波）/CaptureSpeed（去极值估算转速）_19/Step04_按每转三脉冲计算转速 ==
  note: 第四步：将剩余间隔总和换算成每分钟转数
      |
      | 输入有效间隔数n与前一步给出的安全分母S。先求剩余条数n-2，再计算：
      | 转速=60000000×(n-2)/(3×S)。
      |
      | 60000000是一分钟的微秒数；3表示本工程每转3个脉冲；S/(n-2)相当于去极值后的平均脉冲间隔。这
      | 里没有另外的隐含乘100或除100。
      |
      | 例：n=10、S=8000微秒，得到20000转/分。这个数是捕获候选转速，最终仍由外层的数量判断、超时判
      | 断和来源选择决定是否使用。不能因为采用了安全分母就忽略Valid。
  输入1_有效间隔条数 : Inport
  输入2_用于计算的安全分母 : Inport  Port=2
  Add（加减运算）_466 : Sum  Inputs=+-  SaturateOnIntegerOverflow=on  OutDataTypeStr=Inherit: Same as first input
  Cast（数据类型转换）_464 : DataTypeConversion  OutDataTypeStr=single  RndMeth=Round
  Constant（常量）_463 : Constant  Value=60000000  OutDataTypeStr=single
  Constant（常量）_465 : Constant  Value=2  OutDataTypeStr=single
  Constant（常量）_468 : Constant  Value=3  OutDataTypeStr=single
  Numerator（每分钟微秒数乘剩余间隔数）_467 : Product  Inputs=**  SaturateOnIntegerOverflow=on  OutDataTypeStr=Inherit: Same as first input
  Pulses（每转三个脉冲）_469 : Product  Inputs=**  SaturateOnIntegerOverflow=on  OutDataTypeStr=Inherit: Same as first input
  Speed（去极值估算的转速）_470 : Product  Inputs=*/  SaturateOnIntegerOverflow=on  OutDataTypeStr=Inherit: Same as first input
  输出1_捕获候选转速_RPM : Outport
  wires:
  Speed（去极值估算的转速）_470/1 -> 输出1_捕获候选转速_RPM/1
  Pulses（每转三个脉冲）_469/1 -> Speed（去极值估算的转速）_470/2
  Numerator（每分钟微秒数乘剩余间隔数）_467/1 -> Speed（去极值估算的转速）_470/1
  Constant（常量）_468/1 -> Pulses（每转三个脉冲）_469/2
  输入2_用于计算的安全分母/1 -> Pulses（每转三个脉冲）_469/1
  Add（加减运算）_466/1 -> Numerator（每分钟微秒数乘剩余间隔数）_467/2
  Constant（常量）_463/1 -> Numerator（每分钟微秒数乘剩余间隔数）_467/1
  输入1_有效间隔条数/1 -> Cast（数据类型转换）_464/1
  Constant（常量）_465/1 -> Add（加减运算）_466/2
  Cast（数据类型转换）_464/1 -> Add（加减运算）_466/1

== system turbo_controller/BoardOutput_串口封装与阀门时序/Out01_Pump（泵反馈解析与滤波）/Receive（逐字节组帧与保持有效结果）_680/Step01_取字节与循环控制 ==
  note: 第一步：只处理本批收到的字节
      |
      | 接收数组最多64项，Count是这次新收到的数量，Loop给出从1开始的Index。Byte=Rx(Index)，Active=
      | (Index≤Count)。
      |
      | 处理到Index≥Count或Index=64，就把下一循环序号设65，使Loop退出；否则下一序号=Index+1。Coun
      | t=3只处理第1～3项；Count=0时仍走一次无效项保持路径，但不会把数组旧值加入帧。
      |
      | 输出Byte和Active给组帧步骤，下一序号反馈Loop。这里不识别帧头，不作CRC，不把Index当作跨批收
      | 帧位置。
  输入1_本批循环序号 : Inport
  输入2_本批有效字节数 : Inport  Port=2
  输入3_本批接收数组 : Inport  Port=3
  Active（本项在有效范围内）_560 : RelationalOperator  Operator=<=  OutDataTypeStr=boolean  RndMeth=Simplest  InputSameDT=off
  Add（加减运算）_567 : Sum  SaturateOnIntegerOverflow=on  OutDataTypeStr=Inherit: Same as first input
  AtLimit（达到处理上限）_563 : RelationalOperator  Operator===  OutDataTypeStr=boolean  RndMeth=Simplest  InputSameDT=off
  Constant（常量）_562 : Constant  Value=64  OutDataTypeStr=uint32
  Constant（常量）_565 : Constant  Value=65  OutDataTypeStr=uint32
  Constant（常量）_566 : Constant  OutDataTypeStr=uint32
  CurrentByte（按接收顺序取字节）_569 : Selector  InputPortWidth=64  IndexOptions=Index vector (port)  Indices=1  OutputSizes=1
  Last（本周期最后一项）_564 : Logic  Operator=OR  IconShape=distinctive  AllPortsSameDT=off  OutDataTypeStr=boolean
  NextIndex（处理下一项或结束）_568 : Switch  Criteria=u2 ~= 0  SaturateOnIntegerOverflow=off  InputSameDT=off
  ReceivedAll（已处理所有有效项）_561 : RelationalOperator  OutDataTypeStr=boolean  RndMeth=Simplest  InputSameDT=off
  输出1_本项字节 : Outport
  输出2_本项字节有效 : Outport  Port=2
  输出3_下一循环序号 : Outport  Port=3
  wires:
  NextIndex（处理下一项或结束）_568/1 -> 输出3_下一循环序号/1
  Active（本项在有效范围内）_560/1 -> 输出2_本项字节有效/1
  CurrentByte（按接收顺序取字节）_569/1 -> 输出1_本项字节/1
  Add（加减运算）_567/1 -> NextIndex（处理下一项或结束）_568/3
  Last（本周期最后一项）_564/1 -> NextIndex（处理下一项或结束）_568/2
  Constant（常量）_565/1 -> NextIndex（处理下一项或结束）_568/1
  AtLimit（达到处理上限）_563/1 -> Last（本周期最后一项）_564/2
  ReceivedAll（已处理所有有效项）_561/1 -> Last（本周期最后一项）_564/1
  输入3_本批接收数组/1 -> CurrentByte（按接收顺序取字节）_569/1
  Constant（常量）_562/1 -> AtLimit（达到处理上限）_563/2
  Constant（常量）_566/1 -> Add（加减运算）_567/2
  输入2_本批有效字节数/1 -> ReceivedAll（已处理所有有效项）_561/2, Active（本项在有效范围内）_560/2
  输入1_本批循环序号/1 -> Active（本项在有效范围内）_560/1, Add（加减运算）_567/1, AtLimit（达到处理上限）_563/1, CurrentByte（按接收顺序取字节）_569/2, ReceivedAll（已处理所有有效项）_561/1

== system turbo_controller/BoardOutput_串口封装与阀门时序/Out01_Pump（泵反馈解析与滤波）/Receive（逐字节组帧与保持有效结果）_680/Step02_拼帧并保存半帧 ==
  note: 第二步：跨多次接收保存半帧
      |
      | 将本项字节、有效标志、上次候选缓存和上次收帧Position交给Collect。Collect识别AA55并逐项填满
      | 22字节，具体规则已在其内部再拆成五步。
      |
      | 更新后的缓存和Position经原数据类型转换，送回两条记忆块；所以第一次只收到一半，下一批还能接
      | 着填，不必从头找AA。输出候选帧与“本字节刚收齐”，交第三步校验。
      |
      | 候选缓存不等于已接受结果。即使旧缓存里已经有完整内容，没有本次收齐事件也不能再次接受它。这
      | 里的记忆按原循环节奏推进，没有增加一个额外的采样周期等待。
  输入1_本项字节 : Inport
  输入2_本项字节有效 : Inport  Port=2
  Buffer（跨周期收帧缓存）_570 : UnitDelay  InitialCondition=uint8(zeros(22,1))  SampleTime=-1  HasFrameUpgradeWarning=on
  Collect（帧头识别与缓存推进）_611 : Subsystem  Description=|
      | 逐字节组帧：本页只做“找帧头、存字节、推进位置”
      | 
      | 固定帧长为22字节，帧头是十六进制AA、55。输入为上一份候选缓存、已收字节数Position、本次Byte和本字节有效Active。输出为更新缓存、下一次使用的Position和本次收齐事件Complete。
      | 
      | Position不是本批接收数组的序号：0表示还在找AA，1表示已见AA、正在等55，2～21表示头部已确认、继续收后面的内容。跨调用的记忆由外层Step02保存，本页根据输入计算一次更新。
      | 
      | 按五步看：
      | 1 判断当前是否在等AA或55，以及字节是否匹配。
      | 2 决定这个字节应不应该进入候选缓存。
      | 3 算出本次写入位置Position+1，判断是否达到22。
      | 4 允许写入才更新对应一项，否则保留原缓存。
      | 5 按找头、重同步、收齐和无效字节规则，决定下一位置及Complete。
      | 
      | 例：AA→AA→55时，第二个AA保留继续等55的机会，不当作第二帧头写入；头确认后，后续数据即使也是AA或55，仍按普通数据收下。无效字节不推进位置，也不发收齐事件。
      | 
      | Complete仅表示候选帧刚拼满，不表示校验通过；外面的校验步骤还会检查内容。这里没有重写协议或增加等待时间，五步在同一次字节处理内完成。
  Position（已收到的字节数）_571 : UnitDelay  InitialCondition=uint16(0)  SampleTime=-1  HasFrameUpgradeWarning=on
  Store_uint16（按十六位无符号数保存状态）_537039 : DataTypeConversion  Description=为反馈回路显式指定原程序的状态类型，保持原状态更新节拍。  OutDataTypeStr=uint16  RndMeth=Round
  Store_uint8（按八位无符号数保存状态）_537038 : DataTypeConversion  Description=为反馈回路显式指定原程序的状态类型，保持原状态更新节拍。  OutDataTypeStr=uint8  RndMeth=Round
  输出1_本字节刚收齐 : Outport
  输出2_候选帧缓存 : Outport  Port=2
  wires:
  Collect（帧头识别与缓存推进）_611/3(Complete（本字节组成完整帧）_610) -> 输出1_本字节刚收齐/1  "Collect（帧头识别与缓存推进）"
  Collect（帧头识别与缓存推进）_611/1(Buffer（更新后的帧缓存）_608) -> 输出2_候选帧缓存/1, Store_uint8（按八位无符号数保存状态）_537038/1  "Collect（帧头识别与缓存推进）"
  Collect（帧头识别与缓存推进）_611/2(Position（下次接收位置）_609) -> Store_uint16（按十六位无符号数保存状态）_537039/1  "Collect（帧头识别与缓存推进）"
  Store_uint16（按十六位无符号数保存状态）_537039/1 -> Position（已收到的字节数）_571/1
  输入2_本项字节有效/1 -> Collect（帧头识别与缓存推进）_611/4(Active（当前字节有效）_575)
  输入1_本项字节/1 -> Collect（帧头识别与缓存推进）_611/3(Byte（当前字节）_574)
  Position（已收到的字节数）_571/1 -> Collect（帧头识别与缓存推进）_611/2(Position（已收字节数）_573)
  Buffer（跨周期收帧缓存）_570/1 -> Collect（帧头识别与缓存推进）_611/1(Buffer（上次收帧缓存）_572)
  Store_uint8（按八位无符号数保存状态）_537038/1 -> Buffer（跨周期收帧缓存）_570/1

== system turbo_controller/BoardOutput_串口封装与阀门时序/Out01_Pump（泵反馈解析与滤波）/Receive（逐字节组帧与保持有效结果）_680/Step03_收齐且校验通过才接受 ==
  note: 第三步：刚收齐且CRC通过，才接受新帧
      |
      | Complete表示这一项字节刚把22字节补齐，先按原类型传给Verify触发校验。Verify对第6～20字节计
      | 算CRC16，分别与第21、22字节的高、低校验字节比较。
      |
      | 最后Accepted=Complete AND Verify通过。这样未收齐的数据不会被采用，Verify上一帧保留的通过状
      | 态也不会在没有新Complete时重新接收旧帧。
      |
      | CRC初值、表和覆盖范围保留原设置。校验失败只让本次Accepted为假；后面的保持步骤继续输出上一
      | 有效反馈。本处不作反馈比例换算，不直接生成驱动命令。
  输入1_本字节刚收齐 : Inport
  输入2_候选帧缓存 : Inport  Port=2
  Accepted（本字节完成一帧有效数据）_663 : Logic  IconShape=distinctive  AllPortsSameDT=off  OutDataTypeStr=boolean
  Cast（数据类型转换）_661 : DataTypeConversion  OutDataTypeStr=uint32  RndMeth=Round
  Verify（完整帧校验）_662 : Subsystem  Description=|
      | 实际22字节油泵反馈怎样核对CRC
      | 
      | Collect送来的是候选完整帧，本模块只在Complete有效时执行校验。内部取协议指定的待校验字节段，送CRC16逐字节计算，并取出帧尾携带的两个CRC字节。
      | 
      | 16位计算结果分为高低两部分：高字节=floor(CRC/256)，低字节=bitand(CRC,255)。分别与帧中对应位置比较，两项都一致才给出有效结果。
      | 
      | 比如计算CRC为十六进制1234，协议中的CRC高字节必须是12、低字节必须是34；顺序反过来也不能通过。CRC覆盖范围由本页Selector的固定索引决定，不应把帧头或尾部CRC自身随意加入。
      | 
      | 输出交给Receive，与“这一轮确实刚收齐一帧”共同决定是否更新反馈。不完整或校验错误时，外层保留最近有效结果。
      | 
      | 本实例CRC覆盖第6～20字节，与第21、22字节的CRC比较。
  输出1_本字节接受有效帧 : Outport
  wires:
  Accepted（本字节完成一帧有效数据）_663/1 -> 输出1_本字节接受有效帧/1
  输入2_候选帧缓存/1 -> Verify（完整帧校验）_662/2(Frame（完整候选帧）_614)
  Cast（数据类型转换）_661/1 -> Verify（完整帧校验）_662/1(Complete（完整帧执行一次）_612)
  Verify（完整帧校验）_662/1(Valid（校验是否通过）_660) -> Accepted（本字节完成一帧有效数据）_663/2  "Verify（完整帧校验）"
  输入1_本字节刚收齐/1 -> Cast（数据类型转换）_661/1, Accepted（本字节完成一帧有效数据）_663/1

== system turbo_controller/BoardOutput_串口封装与阀门时序/Out01_Pump（泵反馈解析与滤波）/Receive（逐字节组帧与保持有效结果）_680/Step04_换算反馈并保持有效结果 ==
  note: 第四步：还原泵反馈，只在新有效帧时平滑一次
      |
      | 第6、7字节高位在前，合成原始反馈=高字节×256+低字节。再计算候选滤波值=0.875×旧输出+0.125×原
      | 始反馈。
      |
      | Accepted为真时才采用候选值并更新Pump记忆，否则保持旧值。例如旧输出800、新有效反馈1000，本
      | 次结果825；若接着几个调用没有新有效帧，仍是825，不会反复用旧数据再滤波。
      |
      | 这里是接收反馈，不是油泵目标设定。输出随后用于上位机回传；串口控制命令仍由独立输出路径生成
      | 。
  输入1_候选帧缓存 : Inport
  输入2_本字节接受有效帧 : Inport  Port=2
  Cast（数据类型转换）_666 : DataTypeConversion  OutDataTypeStr=uint16  RndMeth=Round
  Cast（数据类型转换）_668 : DataTypeConversion  OutDataTypeStr=uint16  RndMeth=Round
  Cast（数据类型转换）_674 : DataTypeConversion  OutDataTypeStr=single  RndMeth=Round
  Constant（常量）_669 : Constant  Value=256  OutDataTypeStr=uint16
  Constant（常量）_672 : Constant  Value=0.875  OutDataTypeStr=single
  Constant（常量）_675 : Constant  Value=0.125  OutDataTypeStr=single
  High（原始数值高字节）_665 : Selector  InputPortWidth=22  IndexOptions=Index vector (dialog)  Indices=6  OutputSizes=1
  HoldOrUpdate（无有效帧时保持上次反馈）_678 : Switch  Criteria=u2 ~= 0  SaturateOnIntegerOverflow=off  InputSameDT=off
  LowPass（旧值乘0点875加新值乘0点125）_677 : Sum  SaturateOnIntegerOverflow=on  OutDataTypeStr=Inherit: Same as first input
  Low（原始数值低字节）_667 : Selector  InputPortWidth=22  IndexOptions=Index vector (dialog)  Indices=7  OutputSizes=1
  Multiply（相乘）_670 : Product  Inputs=**  SaturateOnIntegerOverflow=on  OutDataTypeStr=Inherit: Same as first input
  Multiply（相乘）_673 : Product  Inputs=**  SaturateOnIntegerOverflow=on  OutDataTypeStr=Inherit: Same as first input
  Multiply（相乘）_676 : Product  Inputs=**  SaturateOnIntegerOverflow=on  OutDataTypeStr=Inherit: Same as first input
  Pump（保持滤波后的油泵转速）_664 : UnitDelay  InitialCondition=single(0)  SampleTime=-1  HasFrameUpgradeWarning=on
  Raw16（合成十六位原始数值）_671 : Sum  SaturateOnIntegerOverflow=on  OutDataTypeStr=Inherit: Same as first input
  Store_single（按单精度数保存状态）_537044 : DataTypeConversion  Description=为反馈回路显式指定原程序的状态类型，保持原状态更新节拍。  OutDataTypeStr=single  RndMeth=Round
  输出1_最近有效反馈 : Outport
  wires:
  HoldOrUpdate（无有效帧时保持上次反馈）_678/1 -> 输出1_最近有效反馈/1, Store_single（按单精度数保存状态）_537044/1
  Cast（数据类型转换）_668/1 -> Raw16（合成十六位原始数值）_671/2
  Multiply（相乘）_670/1 -> Raw16（合成十六位原始数值）_671/1
  Store_single（按单精度数保存状态）_537044/1 -> Pump（保持滤波后的油泵转速）_664/1
  Constant（常量）_675/1 -> Multiply（相乘）_676/2
  Cast（数据类型转换）_674/1 -> Multiply（相乘）_676/1
  Constant（常量）_672/1 -> Multiply（相乘）_673/2
  Constant（常量）_669/1 -> Multiply（相乘）_670/2
  Cast（数据类型转换）_666/1 -> Multiply（相乘）_670/1
  Multiply（相乘）_676/1 -> LowPass（旧值乘0点875加新值乘0点125）_677/2
  Multiply（相乘）_673/1 -> LowPass（旧值乘0点875加新值乘0点125）_677/1
  Pump（保持滤波后的油泵转速）_664/1 -> Multiply（相乘）_673/1, HoldOrUpdate（无有效帧时保持上次反馈）_678/3
  输入2_本字节接受有效帧/1 -> HoldOrUpdate（无有效帧时保持上次反馈）_678/2
  LowPass（旧值乘0点875加新值乘0点125）_677/1 -> HoldOrUpdate（无有效帧时保持上次反馈）_678/1
  输入1_候选帧缓存/1 -> High（原始数值高字节）_665/1, Low（原始数值低字节）_667/1
  Raw16（合成十六位原始数值）_671/1 -> Cast（数据类型转换）_674/1
  Low（原始数值低字节）_667/1 -> Cast（数据类型转换）_668/1
  High（原始数值高字节）_665/1 -> Cast（数据类型转换）_666/1

== system turbo_controller/BoardOutput_串口封装与阀门时序/Out04_Command（电机及油泵指令）/MotorFrame（电机指令高字节固定为零）_925/CRC16（只校验两个命令字节）_912 ==
  note: 【中文学习说明：CRC16查表法】
      | 一、大白话：把逐位算出的答案预先放进表里。
      | 收到每个字节后，用旧校验值和当前字节算一个表下标，
      | 直接查出结果，再与旧值左移一个字节后的部分异或。
      | 每字节只查一次表，不再进行8次逐位循环。
      |
      | 二、本模块一次处理2个数据字节。
      | 每帧校验值从0开始；逐字节循环仍按输入顺序执行。
      | 先将当前字节放到高八位，与旧CRC异或，
      | 再交给TableStep（查表更新）算出新CRC，
      | 记住新CRC后处理下一个字节，最后输出16位结果。
      |
      | 三、和参考工程逐项对应。
      | 参考写法：index=((旧CRC>>8) XOR 当前字节) AND 255。
      | 新CRC=表[index] XOR ((旧CRC<<8) AND 65535)。
      | 本图先合并字节再取高八位，得到完全相同的index。
      | 表为参考工程crc.c中的原始256项uint16数据，
      | 保存在模型工作区CRC16_Table_Reference中，
      | 所有CRC16模块使用同一份表，无需额外源文件。
      |
      | 四、协议规则没有改变。
      | 初值0、多项式0x1021、高位先处理、不作末尾异或。
      | 校验范围由外层选取，帧头和帧尾校验字节不随意加入。
      | 输出仍由外层拆成高、低字节，高字节在前。
      | 这里只计算CRC，是否采纳数据由外层校验比较决定。
      |
      | 五、记忆与循环要分清。
      | 外层逐字节循环在一次调用内处理整段数据，
      | 并非每处理一字节就等待一个采样周期。
      | CRC记忆块传递同一帧中上一个字节的结果；
      | 每次重新计算一帧时从0开始，不串用上一帧的结果。
      | 查表能发现传输错误，不能修复数据，也不是加密。
  note: 整段字节如何逐个累积CRC16
      |
      | 这里的输入Bytes是发给外设的两个命令字节，不含前五项帧头。CRC的作用是把整段字节压缩成一个16
      | 位检查值，便于接收方发现传输内容变化。
      |
      | 每帧从初始CRC=uint16(0)开始。循环一次取一个字节，把该字节乘256移到高8位，与旧CRC异或，得到
      | Merged，再交给TableStep执行查表移位。TableStep的输出成为处理下一个字节的旧CRC。
      |
      | 公式第一步是Merged=bitxor(旧CRC,当前字节×256)。整个循环结束后输出最后一次CRC，父级拆成高、
      | 低字节用于比较或发送。For Iterator中的CRC记忆是帧内累积状态，不能理解成跨帧无限累加。
      |
      | 这里用的是CRC16_Table_Reference指定的算法表，不能随意换另一种CRC表或初始值。相同字节、顺序
      | 、表和初值必须得到相同结果，双方才能校验通过。
  Bytes（待校验字节）_882 : Inport  OutDataTypeStr=uint8
  CRC（本帧累计校验值）_884 : UnitDelay  InitialCondition=uint16(0)  SampleTime=-1  HasFrameUpgradeWarning=on
  Cast（数据类型转换）_886 : DataTypeConversion  OutDataTypeStr=uint16  RndMeth=Round
  Constant（常量）_887 : Constant  Value=256  OutDataTypeStr=uint16
  CurrentByte（当前字节）_885 : Selector  InputPortWidth=2  IndexOptions=Index vector (port)  Indices=1  OutputSizes=1
  EachByte（逐字节校验）_883 : ForIterator  ResetStates=reset  IterationLimit=2  IterationVariableDataType=uint32
  HighByte（字节移到高八位）_888 : Product  Inputs=**  SaturateOnIntegerOverflow=on  OutDataTypeStr=Inherit: Same as first input
  MergeByte（并入一个字节）_889 : simulink/Logic and Bit Operations/Bitwise Operator  logicop=XOR  UseBitMask=off  NumInputPorts=2  BitMask=bin2dec('11011001')  BitMaskRealWorld=Stored Integer
      settings: LibrarySourceBlock=|
      | hdlsllib/Logic and Bit
      | Operations/Bitwise
      | Operator
  Store_uint16（按十六位无符号数保存状态）_537380 : DataTypeConversion  Description=为反馈回路显式指定原程序的状态类型，保持原状态更新节拍。  OutDataTypeStr=uint16  RndMeth=Round
  TableStep（查表更新本字节校验） : Subsystem  Description=|
      | CRC16的一个字节怎样查表更新
      | 
      | 父级已经把当前数据字节异或进旧CRC的高8位，形成Merged。本模块把这个16位数拆成“用哪项表”和“保留哪些移位结果”两部分。
      | 
      | 先取高8位：索引=floor(Merged/256)，范围0～255。用它到CRC16_Table_Reference查表；模型Selector按零基索引取值，写成MATLAB数组下标时要用索引+1。
      | 另一条支路把Merged左移一个字节，即乘256，然后只保留低16位：移位值=bitand(uint32(Merged)×256,65535)。
      | 
      | 最后将表值与移位值按位异或：
      | 新CRC=bitxor(表值,移位值)。
      | 
      | 例如Merged=十六进制1234，高8位12用于选表项，左移并截16位后为3400，再与表项异或。宽类型uint32是为了中间计算不先溢出，并不表示输出CRC变成32位。结果回到父级，继续处理下一个数据字节。
  CRC16（本帧校验结果）_911 : Outport
  wires:
  Constant（常量）_887/1 -> HighByte（字节移到高八位）_888/2  "Constant（常量）"
  Cast（数据类型转换）_886/1 -> HighByte（字节移到高八位）_888/1  "Cast（数据类型转换）"
  CurrentByte（当前字节）_885/1 -> Cast（数据类型转换）_886/1  "CurrentByte（当前字节）"
  EachByte（逐字节校验）_883/1 -> CurrentByte（当前字节）_885/2  "EachByte（逐字节校验）"
  Bytes（待校验字节）_882/1 -> CurrentByte（当前字节）_885/1  "Bytes（待校验字节）"
  TableStep（查表更新本字节校验）/1(CRC（本字节处理后的校验值）) -> CRC16（本帧校验结果）_911/1, Store_uint16（按十六位无符号数保存状态）_537380/1  "CRC16（查表更新结果）"
  MergeByte（并入一个字节）_889/1 -> TableStep（查表更新本字节校验）/1(Merged（旧校验值与当前字节异或后的数）)  "Merged（旧CRC与当前字节合并值）"
  HighByte（字节移到高八位）_888/1 -> MergeByte（并入一个字节）_889/2  "HighByte（字节移到高八位）"
  CRC（本帧累计校验值）_884/1 -> MergeByte（并入一个字节）_889/1  "CRC（本帧累计校验值）"
  Store_uint16（按十六位无符号数保存状态）_537380/1 -> CRC（本帧累计校验值）_884/1
